simulink model "Gyroscope"  (R2026a)
settings: Solver=VariableStepAuto
values from neighbouring files (symbols this model uses):
  Bias_static = [1.8; -1.8; 1.8] * (1/3600) * (pi/180)    [gyro.m]
  M_misalign = [1,  g_xy,  g_xz ... (first row only)    [gyro.m]
  Scale_factor = [500; -450; 300]    [gyro.m]
  Ts = 0.01    [gyro.m]
undefined symbols (not defined in the file or in its folder): DiscIntNeverNeededParam
libraries: simulink x2
settings Model: Creator=romas  LastModifiedBy=romas

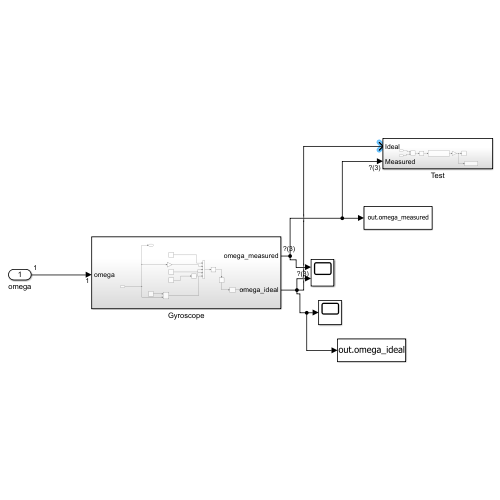
[thumbnail: Simulink's stored preview of the top-level diagram]
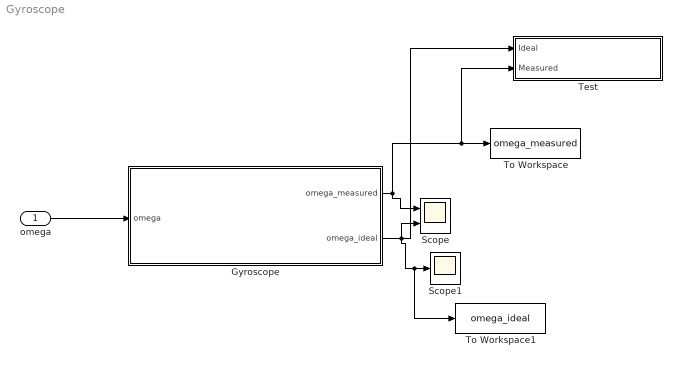
== system Gyroscope ==
  omega : Inport
  Gyroscope : Subsystem
  Scope : Scope  NumInputPorts=2
      settings: ActiveDisplayYMinimum=-0.00607589525  ActiveDisplayYMaximum=0.0058140972500000006
  Scope1 : Scope
      settings: ActiveDisplayYMinimum=-0.004344809437227053  ActiveDisplayYMaximum=0.0039028388290876471
  Test : Subsystem
  To Workspace : ToWorkspace  VariableName=omega_measured  SampleTime=-1
      settings: Save2DSignal=2-D array (concatenate along first dimension)
  To Workspace1 : ToWorkspace  VariableName=omega_ideal  SampleTime=-1
      settings: Save2DSignal=2-D array (concatenate along first dimension)
  wires:
  Gyroscope/2(omega_ideal) -> Test/1(Ideal), To Workspace1/1, Scope1/1, Scope/2
  omega/1 -> Gyroscope/1(omega)
  Gyroscope/1(omega_measured) -> Scope/1, Test/2(Measured), To Workspace/1

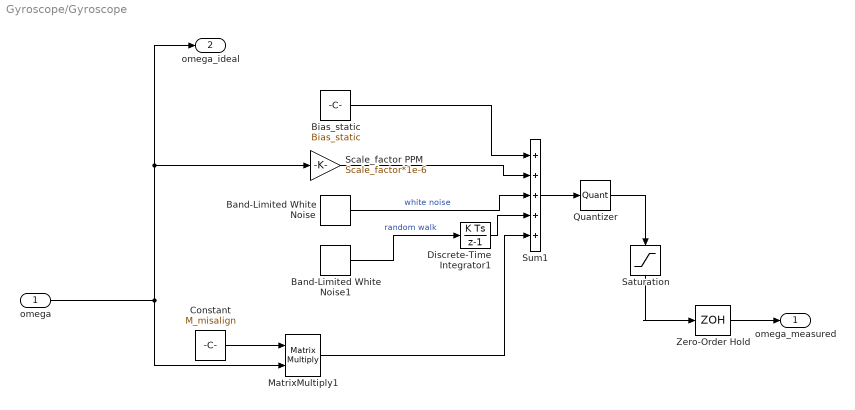
== system Gyroscope/Gyroscope ==
  omega : Inport
  Band-Limited White Noise : simulink/Sources/Band-Limited White Noise  Cov=[1.218e-9; 1.218e-9; 1.218e-9]  Ts=Ts  seed=[23; 42; 101]
  Band-Limited White Noise1 : simulink/Sources/Band-Limited White Noise  Cov=[9.39e-14; 9.39e-14; 9.39e-14]  Ts=Ts  seed=[76; 1240; 3550]
  Bias_static : Constant  Value=Bias_static
  Constant : Constant  Value=M_misalign
  Discrete-Time Integrator1 : DiscreteIntegrator  SampleTime=-1  ICPrevOutput=DiscIntNeverNeededParam  ICPrevScaledInput=DiscIntNeverNeededParam
  MatrixMultiply1 : Product  Multiplication=Matrix(*)
  Quantizer : Quantizer  QuantizationInterval=8.7266e-5
  Saturation : Saturate  UpperLimit=2000  LowerLimit=-2000
  Scale_factor PPM : Gain  Gain=Scale_factor*1e-6
  Sum1 : Sum  Inputs=+++++
  Zero-Order Hold : ZeroOrderHold  SampleTime=-1
  omega_measured : Outport
  omega_ideal : Outport  Port=2
  wires:
  Zero-Order Hold/1 -> omega_measured/1
  Band-Limited White Noise/1 -> Sum1/3  "white noise"
  Band-Limited White Noise1/1 -> Discrete-Time Integrator1/1  "random walk"
  Scale_factor PPM/1 -> Sum1/2
  Sum1/1 -> Quantizer/1
  Quantizer/1 -> Saturation/1
  Saturation/1 -> Zero-Order Hold/1
  Bias_static/1 -> Sum1/1
  omega/1 -> omega_ideal/1, Scale_factor PPM/1, MatrixMultiply1/2
  Discrete-Time Integrator1/1 -> Sum1/4
  Constant/1 -> MatrixMultiply1/1
  MatrixMultiply1/1 -> Sum1/5

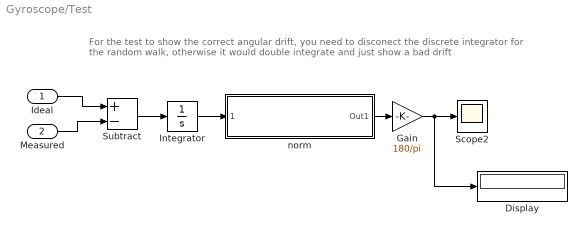
== system Gyroscope/Test ==
  note: For the test to show the correct angular drift, you need to disconect the discrete integrator for the random walk, otherwise it would double integrate and just show a bad drift
  Ideal : Inport
  Measured : Inport  Port=2
  Display : Display
  Gain : Gain  Gain=180/pi
  Integrator : Integrator
  Scope2 : Scope
      settings: ActiveDisplayYMinimum=-4.2395030543025944  ActiveDisplayYMaximum=38.155527488723358  DataLoggingVariableName=ScopeData3
  Subtract : Sum  Inputs=+-
  norm : Subsystem
  wires:
  Ideal/1 -> Subtract/1
  Measured/1 -> Subtract/2
  Subtract/1 -> Integrator/1
  Integrator/1 -> norm/1(1)
  Gain/1 -> Display/1, Scope2/1
  norm/1(Out1) -> Gain/1

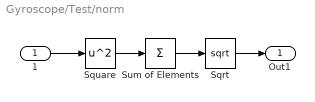
== system Gyroscope/Test/norm ==
  1 : Inport
  Sqrt : Sqrt
  Square : Math  Operator=square
  Sum of Elements : Sum  Inputs=+
  Out1 : Outport
  wires:
  Sqrt/1 -> Out1/1
  Sum of Elements/1 -> Sqrt/1
  Square/1 -> Sum of Elements/1
  1/1 -> Square/1
